simulink model "Longitidunal_Vehicle_Dynamics"  (R2025b)
settings: Solver=ode8  StartTime=0.0  StopTime=200  FixedStep=0.01  RelTol=1e-3
InitFcn:
  | cx=0.32;
  | A=2; %m^2
  | ro=1.22; %kg/m^3
  | r=(15*0.0254)/2+(0.185*0.65); %m
  | rw=0.98*r; %Effectiveradius
  | m=1200; %kg
  | g=9.81; %m/s^2
  | l=2.4; %m
  | a1=1.1; %m
  | a2=1.4; %m
  | h=0.0508; %m
  | mu0=0.015; %Jazar
  | mu1=7e-6; %Jazar
  | mu=0.8; %Jazar
  | teta=0;
  | J_w=1.2; %kg/m^2
  | Iz=3000; %kg/m^2
  | Calfaf=75000; %N/rad
  | Calfar=75000; %N/rad
  | ms=375; %Jazar
  | cs=1200; %Jazar
  | ks=35000; %Jazar
  | mu=75; %Jazar
  | cu=0; %Jazar
  | ku=193000; %
settings Model: Creator=xps  LastModifiedBy=MehrSystem
settings SolverCC: ZeroCrossAlgorithm=Adaptive  AlgebraicLoopSolver=TrustRegion
settings DataIOCC: ReturnWorkspaceOutputs=off
settings OptimizationCC: DefaultParameterBehavior=Inlined  OptimizeBlockIOStorage=off  BufferReuse=off  ReuseModelBlockBuffer=off  GlobalBufferReuse=off  ExpressionFolding=off  EnableMemcpy=off  PassReuseOutputArgsAs=Individual arguments  LocalBlockOutputs=off  ZeroExternalMemoryAtStartup=off  ZeroInternalMemoryAtStartup=off  OptimizeDataStoreBuffers=off  BusAssignmentInplaceUpdate=off  OptimizationLevel=level0  OptimizationCustomize=off  EfficientTunableParamExpr=on
settings DebuggingCC: MaxConsecutiveZCsMsg=none  ParameterTunabilityLossMsg=error  UnconnectedInputMsg=warning  UnconnectedOutputMsg=warning  UnconnectedLineMsg=warning  ArithmeticOperatorsInVariantConditions=warning
settings ModelReferenceCC: EnableRefExpFcnMdlSchedulingChecks=on
settings SFSimCC: SimUseLocalCustomCode=off  MATLABDynamicMemAlloc=off  CustomCodeUndefinedFunction=UseInterfaceOnly
settings RTWCC: SystemTargetFile=ert.tlc  TemplateMakefile=ert_default_tmf  RTWUseLocalCustomCode=off  GPUComputeCapability=3.5  Description=Embedded Coder
settings CodeAppCC: ForceParamTrailComments=on  IgnoreCustomStorageClasses=off  OperatorAnnotations=on  SimulinkDataObjDesc=on  SFDataObjDesc=on  InsertBlockDesc=on
settings ERTTargetCC: ERTCustomFileTemplate=example_file_process.tlc  TargetLangStandard=C99 (ISO)  GenerateSampleERTMain=on  SupportContinuousTime=on

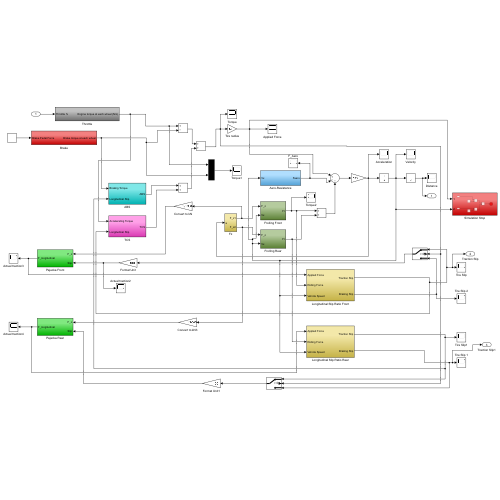
[thumbnail: Simulink's stored preview of the top-level diagram]
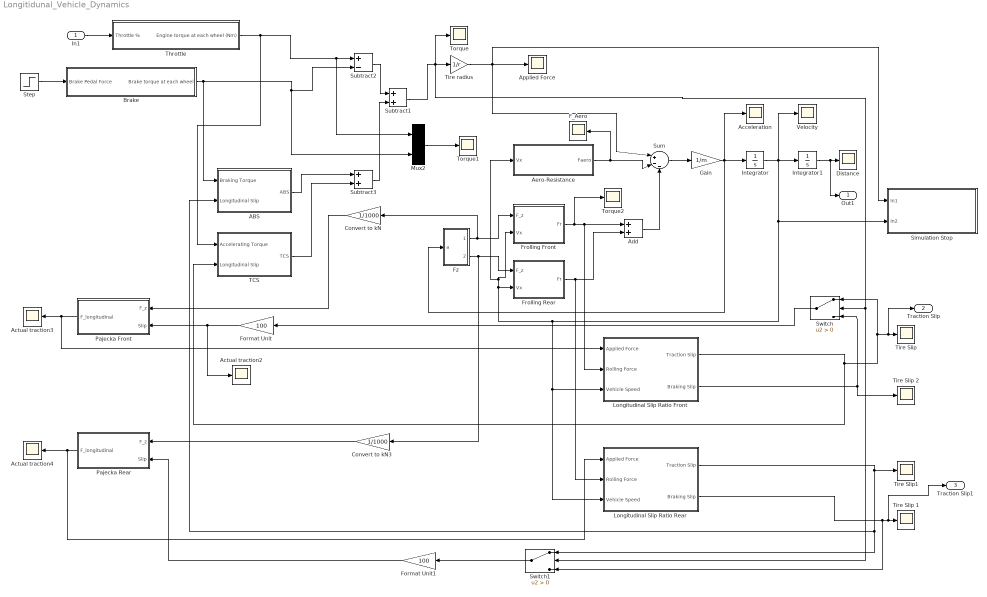
== system Longitidunal_Vehicle_Dynamics ==
  In1 : Inport
  ABS : Subsystem
  Acceleration : Scope
      settings: ActiveDisplayYMinimum=-11.20211075688924  ActiveDisplayYMaximum=1.1595227229876932  DataLoggingVariableName=ScopeData2
  Actual traction2 : Scope
      settings: ActiveDisplayYMinimum=-9.6127540741225162E+14  ActiveDisplayYMaximum=2.5798371932340445E+15  DataLoggingVariableName=ScopeData3
  Actual traction3 : Scope
      settings: ActiveDisplayYMinimum=-2781.3956583754534  ActiveDisplayYMaximum=-2659.1708426364712  DataLoggingVariableName=ScopeData5
  Actual traction4 : Scope
      settings: ActiveDisplayYMinimum=-2116.02176137597  ActiveDisplayYMaximum=-1996.3163945739989  DataLoggingVariableName=ScopeData2
  Add : Sum
  Aero-Resistance : Subsystem
  Applied Force : Scope
      settings: ActiveDisplayYMinimum=-7916.33146  ActiveDisplayYMaximum=1737.7313  DataLoggingVariableName=ScopeData6
  Brake : Subsystem
  Convert to kN : Gain  Gain=1/1000
  Convert to kN3 : Gain  Gain=1/1000
  Distance : Scope
      settings: ActiveDisplayYMinimum=-2186.3043007629622  ActiveDisplayYMaximum=242.92270008477351
  F_Aero : Scope
      settings: ActiveDisplayYMinimum=-66.76965  ActiveDisplayYMaximum=600.92681
  Format Unit : Gain  Gain=100
  Format Unit1 : Gain  Gain=100
  Frolling Front : Subsystem
  Frolling Rear : Subsystem
  Fz : Subsystem
  Gain : Gain  Gain=1/m
  Integrator : Integrator
  Integrator1 : Integrator
  Longitudinal Slip Ratio Front : Subsystem
  Longitudinal Slip Ratio Rear : Subsystem
  Mux2 : Mux  Inputs=2
  Pajecka Front : Subsystem
  Pajecka Rear : Subsystem
  Simulation Stop : Subsystem
  Step : Step  Time=120  After=30  SampleTime=0
  Subtract1 : Sum
  Subtract2 : Sum  Inputs=+-
  Subtract3 : Sum
  Sum : Sum  Inputs=|+--
  Switch : Switch  Criteria=u2 > Threshold  SaturateOnIntegerOverflow=off  InputSameDT=off
  Switch1 : Switch  Criteria=u2 > Threshold  SaturateOnIntegerOverflow=off  InputSameDT=off
  TCS : Subsystem
  Throttle : Subsystem
  Tire Slip : Scope
      settings: ActiveDisplayYMinimum=0.99985  ActiveDisplayYMaximum=1.00139  DataLoggingVariableName=ScopeData2
  Tire Slip 1 : Scope
      settings: ActiveDisplayYMinimum=-592.75065171892868  ActiveDisplayYMaximum=58.517501440809937  DataLoggingVariableName=ScopeData6
  Tire Slip 2 : Scope
      settings: ActiveDisplayYMinimum=-1469.7388232940821  ActiveDisplayYMaximum=-771.732664711504  DataLoggingVariableName=ScopeData3
  Tire Slip1 : Scope
      settings: ActiveDisplayYMinimum=0.98434  ActiveDisplayYMaximum=1.14093  DataLoggingVariableName=ScopeData7
  Tire radius : Gain  Gain=1/r
  Torque : Scope
      settings: ActiveDisplayYMinimum=-220  ActiveDisplayYMaximum=-20  DataLoggingVariableName=ScopeData5
  Torque1 : Scope
      settings: ActiveDisplayYMinimum=-75  ActiveDisplayYMaximum=675
  Torque2 : Scope
      settings: ActiveDisplayYMinimum=33.8504  ActiveDisplayYMaximum=141.74668  DataLoggingVariableName=ScopeData2
  Velocity : Scope
      settings: ActiveDisplayYMinimum=-4.60487  ActiveDisplayYMaximum=41.44379
  Out1 : Outport
  Traction Slip : Outport  Port=2
  Traction Slip1 : Outport  Port=3
  wires:
  Gain/1 -> Fz/1(a), Acceleration/1, Integrator/1
  Integrator/1 -> Simulation Stop/2(In2), Longitudinal Slip Ratio Rear/3(Vehicle Speed), Longitudinal Slip Ratio Front/3(Vehicle Speed), Aero-Resistance/1(Vx), Frolling Front/2(Vx), Frolling Rear/2(Vx), Velocity/1, Integrator1/1
  Sum/1 -> Gain/1
  Aero-Resistance/1(Faero) -> F_Aero/1, Sum/2
  Fz/1(F_z1) -> Convert to kN/1, Frolling Front/1(F_z)
  Fz/2(F_z2) -> Convert to kN3/1, Frolling Rear/1(F_z)
  Frolling Front/1(Fr) -> Torque2/1, Longitudinal Slip Ratio Front/2(Rolling Force), Add/1
  Add/1 -> Sum/3
  Subtract1/1 -> Torque/1, Switch/2, Switch1/2, Tire radius/1
  Throttle/1(Engine torque at each wheel (Nm)) -> TCS/1(Accelerating Torque), Subtract2/1, Mux2/1
  Brake/1(Brake torque at each wheel) -> Subtract2/2, Mux2/2, ABS/1(Braking Torque)
  Integrator1/1 -> Out1/1, Distance/1
  Convert to kN/1 -> Pajecka Front/1(F_z)
  Format Unit/1 -> Pajecka Front/2(Slip), Actual traction2/1
  Longitudinal Slip Ratio Front/1(Traction Slip) -> TCS/2(Longitudinal Slip), Switch/1, Traction Slip/1, Tire Slip/1
  Longitudinal Slip Ratio Front/2(Braking Slip) -> Switch/3, Tire Slip 2/1
  Longitudinal Slip Ratio Rear/2(Braking Slip) -> Switch1/3, Traction Slip1/1, Tire Slip 1/1
  Convert to kN3/1 -> Pajecka Rear/1(F_z)
  Longitudinal Slip Ratio Rear/1(Traction Slip) -> ABS/2(Longitudinal Slip), Switch1/1, Tire Slip1/1
  Pajecka Rear/1(F_longitudinal) -> Longitudinal Slip Ratio Rear/1(Applied Force), Actual traction4/1
  Switch/1 -> Format Unit/1
  Switch1/1 -> Format Unit1/1
  Mux2/1 -> Torque1/1
  In1/1 -> Throttle/1(Throttle %)
  Format Unit1/1 -> Pajecka Rear/2(Slip)
  Tire radius/1 -> Simulation Stop/1(In1), Sum/1, Applied Force/1
  Step/1 -> Brake/1(Brake Pedal Force)
  Pajecka Front/1(F_longitudinal) -> Actual traction3/1, Longitudinal Slip Ratio Front/1(Applied Force)
  Subtract2/1 -> Subtract1/1
  Frolling Rear/1(Fr) -> Longitudinal Slip Ratio Rear/2(Rolling Force), Add/2
  TCS/1(TCS) -> Subtract3/2
  ABS/1(ABS) -> Subtract3/1
  Subtract3/1 -> Subtract1/2

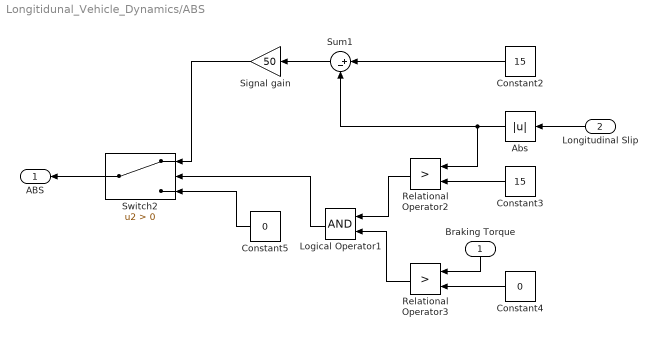
== system Longitidunal_Vehicle_Dynamics/ABS ==
  Braking Torque : Inport
  Longitudinal Slip : Inport  Port=2
  Abs : Abs  SaturateOnIntegerOverflow=off
  Constant2 : Constant  Value=15
  Constant3 : Constant  Value=15
  Constant4 : Constant  Value=0
  Constant5 : Constant  Value=0
  Logical Operator1 : Logic  AllPortsSameDT=off  OutDataTypeStr=boolean
  Relational Operator2 : RelationalOperator  Operator=>  OutDataTypeStr=boolean  RndMeth=Simplest  InputSameDT=off
  Relational Operator3 : RelationalOperator  Operator=>  OutDataTypeStr=boolean  RndMeth=Simplest  InputSameDT=off
  Signal gain : Gain  Gain=50
  Sum1 : Sum  Inputs=|+-
  Switch2 : Switch  Criteria=u2 > Threshold  SaturateOnIntegerOverflow=off  InputSameDT=off
  ABS : Outport  VectorParamsAs1DForOutWhenUnconnected=off
  wires:
  Sum1/1 -> Signal gain/1
  Constant4/1 -> Relational Operator3/2
  Longitudinal Slip/1 -> Abs/1
  Braking Torque/1 -> Relational Operator3/1
  Switch2/1 -> ABS/1
  Relational Operator2/1 -> Logical Operator1/1
  Constant3/1 -> Relational Operator2/2
  Logical Operator1/1 -> Switch2/2
  Constant2/1 -> Sum1/1
  Relational Operator3/1 -> Logical Operator1/2
  Constant5/1 -> Switch2/3
  Abs/1 -> Relational Operator2/1, Sum1/2
  Signal gain/1 -> Switch2/1

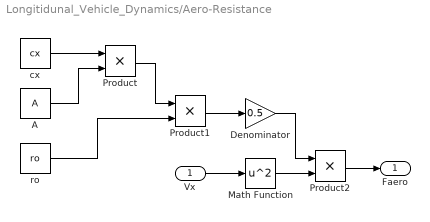
== system Longitidunal_Vehicle_Dynamics/Aero-Resistance ==
  Vx : Inport
  A : Constant  Value=A
  Denominator : Gain  Gain=0.5
  Math Function : Math  Operator=square  SignedPower=on
  Product : Product
  Product1 : Product
  Product2 : Product
  cx : Constant  Value=cx
  ro : Constant  Value=ro
  Faero : Outport  VectorParamsAs1DForOutWhenUnconnected=off
  wires:
  A/1 -> Product/2
  Product1/1 -> Denominator/1
  Denominator/1 -> Product2/1
  Vx/1 -> Math Function/1
  Product2/1 -> Faero/1
  ro/1 -> Product1/2
  cx/1 -> Product/1
  Math Function/1 -> Product2/2
  Product/1 -> Product1/1

== system Longitidunal_Vehicle_Dynamics/Brake ==
  Brake Pedal Force : Inport
  Gain : Gain  Gain=400
  Gain1 : Gain
  r_static : Gain  Gain=0.3
  Brake torque at each wheel : Outport  VectorParamsAs1DForOutWhenUnconnected=off
  wires:
  Gain1/1 -> r_static/1
  Gain/1 -> Gain1/1
  Brake Pedal Force/1 -> Gain/1
  r_static/1 -> Brake torque at each wheel/1

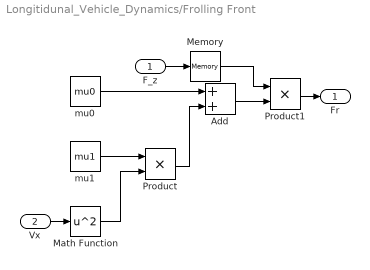
== system Longitidunal_Vehicle_Dynamics/Frolling Front ==
  F_z : Inport
  Vx : Inport  Port=2
  Add : Sum
  Math Function : Math  Operator=square  SignedPower=on
  Memory : Memory
  Product : Product
  Product1 : Product
  mu0 : Constant  Value=mu0
  mu1 : Constant  Value=mu1
  Fr : Outport  VectorParamsAs1DForOutWhenUnconnected=off
  wires:
  Add/1 -> Product1/2
  Math Function/1 -> Product/2
  Product/1 -> Add/2
  mu0/1 -> Add/1
  mu1/1 -> Product/1
  Vx/1 -> Math Function/1
  Product1/1 -> Fr/1
  F_z/1 -> Memory/1
  Memory/1 -> Product1/1

== system Longitidunal_Vehicle_Dynamics/Frolling Rear ==
  F_z : Inport
  Vx : Inport  Port=2
  Add : Sum
  Math Function : Math  Operator=square  SignedPower=on
  Memory : Memory
  Product : Product
  Product1 : Product
  mu0 : Constant  Value=mu0
  mu1 : Constant  Value=mu1
  Fr : Outport  VectorParamsAs1DForOutWhenUnconnected=off
  wires:
  F_z/1 -> Memory/1
  Product1/1 -> Fr/1
  Vx/1 -> Math Function/1
  mu1/1 -> Product/1
  mu0/1 -> Add/1
  Product/1 -> Add/2
  Math Function/1 -> Product/2
  Add/1 -> Product1/2
  Memory/1 -> Product1/1

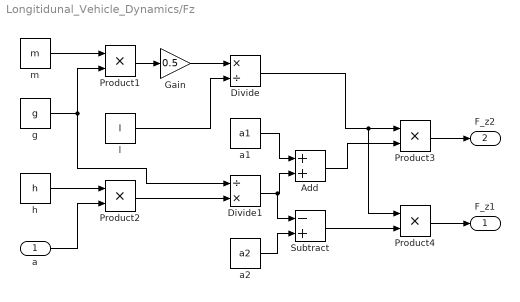
== system Longitidunal_Vehicle_Dynamics/Fz ==
  a : Inport
  Add : Sum
  Divide : Product  Inputs=*/
  Divide1 : Product  Inputs=/*
  Gain : Gain  Gain=0.5
  Product{1..4} (4 alike) : Product
  Subtract : Sum  Inputs=-+
  a1 : Constant  Value=a1
  a2 : Constant  Value=a2
  g : Constant  Value=g
  h : Constant  Value=h
  l : Constant  Value=l
  m : Constant  Value=m
  F_z1 : Outport  VectorParamsAs1DForOutWhenUnconnected=off
  F_z2 : Outport  Port=2  VectorParamsAs1DForOutWhenUnconnected=off
  wires:
  m/1 -> Product1/1
  g/1 -> Divide1/1, Product1/2
  Product1/1 -> Gain/1
  Gain/1 -> Divide/1
  l/1 -> Divide/2
  h/1 -> Product2/1
  Product2/1 -> Divide1/2
  a1/1 -> Add/1
  Divide1/1 -> Subtract/1, Add/2
  Divide/1 -> Product4/1, Product3/1
  Add/1 -> Product3/2
  a2/1 -> Subtract/2
  Subtract/1 -> Product4/2
  Product4/1 -> F_z1/1
  Product3/1 -> F_z2/1
  a/1 -> Product2/2

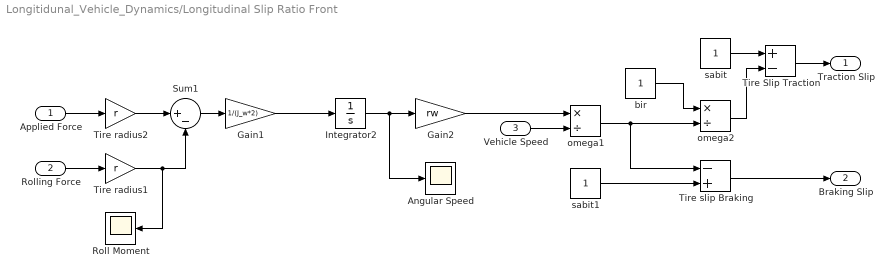
== system Longitidunal_Vehicle_Dynamics/Longitudinal Slip Ratio Front ==
  Applied Force : Inport
  Rolling Force : Inport  Port=2
  Vehicle Speed : Inport  Port=3
  Angular Speed : Scope
      settings: ActiveDisplayYMinimum=-754.25402  ActiveDisplayYMaximum=6788.28715
  Gain1 : Gain  Gain=1/(J_w*2)
  Gain2 : Gain  Gain=rw
  Integrator2 : Integrator  InitialCondition=0.0001
  Roll Moment : Scope
      settings: ActiveDisplayYMinimum=12.74052  ActiveDisplayYMaximum=24.56596  DataLoggingVariableName=ScopeData6
  Sum1 : Sum  Inputs=|+-
  Tire Slip Traction : Sum  Inputs=+-
  Tire radius1 : Gain  Gain=r
  Tire radius2 : Gain  Gain=r
  Tire slip Braking : Sum  Inputs=-+
  bir : Constant
  omega1 : Product  Inputs=*/
  omega2 : Product  Inputs=*/
  sabit : Constant
  sabit1 : Constant
  Traction Slip : Outport  VectorParamsAs1DForOutWhenUnconnected=off
  Braking Slip : Outport  Port=2  VectorParamsAs1DForOutWhenUnconnected=off
  wires:
  Rolling Force/1 -> Tire radius1/1
  Vehicle Speed/1 -> omega1/2
  Tire slip Braking/1 -> Braking Slip/1
  Integrator2/1 -> Gain2/1, Angular Speed/1
  sabit/1 -> Tire Slip Traction/1
  bir/1 -> omega2/1
  omega2/1 -> Tire Slip Traction/2
  Tire Slip Traction/1 -> Traction Slip/1
  Gain1/1 -> Integrator2/1
  Gain2/1 -> omega1/1
  omega1/1 -> Tire slip Braking/1, omega2/2
  Tire radius1/1 -> Sum1/2, Roll Moment/1
  sabit1/1 -> Tire slip Braking/2
  Applied Force/1 -> Tire radius2/1
  Sum1/1 -> Gain1/1
  Tire radius2/1 -> Sum1/1

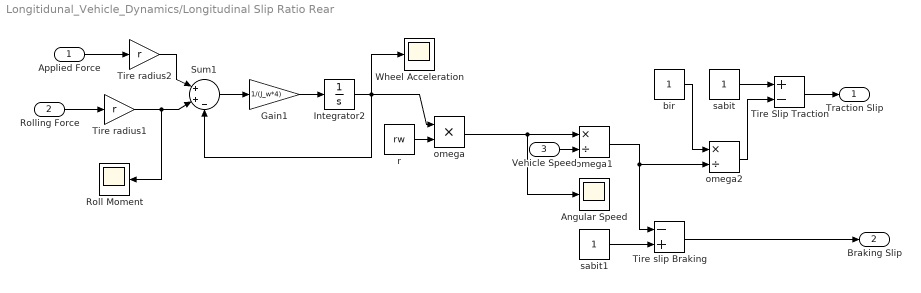
== system Longitidunal_Vehicle_Dynamics/Longitudinal Slip Ratio Rear ==
  Applied Force : Inport
  Rolling Force : Inport  Port=2
  Vehicle Speed : Inport  Port=3
  Angular Speed : Scope
      settings: ActiveDisplayYMinimum=-1  ActiveDisplayYMaximum=1
  Gain1 : Gain  Gain=1/(J_w*4)
  Integrator2 : Integrator  InitialCondition=0.0001
  Roll Moment : Scope
      settings: ActiveDisplayYMinimum=9.72165  ActiveDisplayYMaximum=18.82881  DataLoggingVariableName=ScopeData6
  Sum1 : Sum  Inputs=|++-
  Tire Slip Traction : Sum  Inputs=+-
  Tire radius1 : Gain  Gain=r
  Tire radius2 : Gain  Gain=r
  Tire slip Braking : Sum  Inputs=-+
  Wheel Acceleration : Scope
      settings: ActiveDisplayYMinimum=-31.80693  ActiveDisplayYMaximum=286.2624  DataLoggingVariableName=ScopeData4
  bir : Constant
  omega : Product  Inputs=**
  omega1 : Product  Inputs=*/
  omega2 : Product  Inputs=*/
  r : Constant  Value=rw
  sabit : Constant
  sabit1 : Constant
  Traction Slip : Outport  VectorParamsAs1DForOutWhenUnconnected=off
  Braking Slip : Outport  Port=2  VectorParamsAs1DForOutWhenUnconnected=off
  wires:
  sabit1/1 -> Tire slip Braking/2
  Tire radius1/1 -> Roll Moment/1, Sum1/2
  omega1/1 -> omega2/2, Tire slip Braking/1
  omega/1 -> omega1/1, Angular Speed/1
  r/1 -> omega/2
  Gain1/1 -> Integrator2/1
  Tire Slip Traction/1 -> Traction Slip/1
  omega2/1 -> Tire Slip Traction/2
  bir/1 -> omega2/1
  Sum1/1 -> Gain1/1
  sabit/1 -> Tire Slip Traction/1
  Integrator2/1 -> Sum1/3, Wheel Acceleration/1, omega/1
  Tire slip Braking/1 -> Braking Slip/1
  Vehicle Speed/1 -> omega1/2
  Applied Force/1 -> Tire radius2/1
  Rolling Force/1 -> Tire radius1/1
  Tire radius2/1 -> Sum1/1

== system Longitidunal_Vehicle_Dynamics/Pajecka Front ==
  F_z : Inport
  Slip : Inport  Port=2
  Longitudinal : Subsystem
  Subsystem : Subsystem
  F_longitudinal : Outport  VectorParamsAs1DForOutWhenUnconnected=off
  wires:
  Longitudinal/1(F) -> F_longitudinal/1
  F_z/1 -> Subsystem/1(F_z)
  Slip/1 -> Subsystem/2(slip)
  Subsystem/4(E) -> Longitudinal/3(E)
  Subsystem/5(Bx1) -> Longitudinal/4(Bx1)
  Subsystem/1(C) -> Longitudinal/1(C)
  Subsystem/2(D) -> Longitudinal/2(D)
  Subsystem/3(V) -> Longitudinal/5(V)

== system Longitidunal_Vehicle_Dynamics/Pajecka Rear ==
  F_z : Inport
  Slip : Inport  Port=2
  Longitudinal : Subsystem
  Subsystem : Subsystem
  F_longitudinal : Outport  VectorParamsAs1DForOutWhenUnconnected=off
  wires:
  Longitudinal/1(F) -> F_longitudinal/1
  F_z/1 -> Subsystem/1(F_z)
  Slip/1 -> Subsystem/2(slip)
  Subsystem/4(E) -> Longitudinal/3(E)
  Subsystem/5(Bx1) -> Longitudinal/4(Bx1)
  Subsystem/1(C) -> Longitudinal/1(C)
  Subsystem/2(D) -> Longitudinal/2(D)
  Subsystem/3(V) -> Longitudinal/5(V)

== system Longitidunal_Vehicle_Dynamics/Simulation Stop ==
  In1 : Inport
  In2 : Inport  Port=2
  Constant : Constant  Value=0.1
  Constant1 : Constant  Value=0
  Logical Operator : Logic  AllPortsSameDT=off  OutDataTypeStr=boolean
  Relational Operator : RelationalOperator  Operator=<=  OutDataTypeStr=boolean  RndMeth=Simplest  InputSameDT=off
  Relational Operator1 : RelationalOperator  Operator=<  OutDataTypeStr=boolean  RndMeth=Simplest  InputSameDT=off
  Stop Simulation : Stop
  wires:
  Relational Operator1/1 -> Logical Operator/1
  Relational Operator/1 -> Logical Operator/2
  Constant/1 -> Relational Operator/2
  Constant1/1 -> Relational Operator1/2
  Logical Operator/1 -> Stop Simulation/1
  In2/1 -> Relational Operator/1
  In1/1 -> Relational Operator1/1

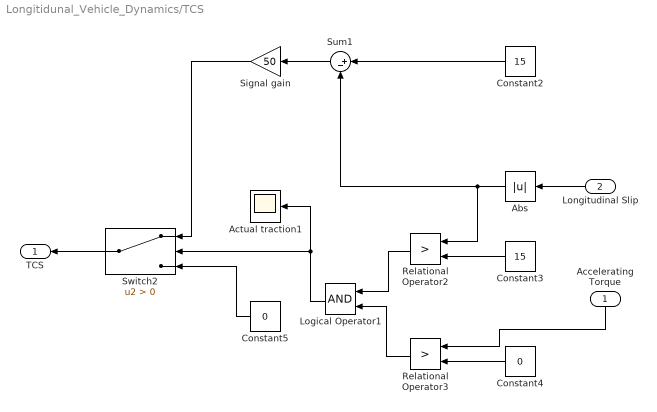
== system Longitidunal_Vehicle_Dynamics/TCS ==
  Accelerating Torque : Inport
  Longitudinal Slip : Inport  Port=2
  Abs : Abs  SaturateOnIntegerOverflow=off
  Actual traction1 : Scope
      settings: ActiveDisplayYMinimum=-1  ActiveDisplayYMaximum=1
  Constant2 : Constant  Value=15
  Constant3 : Constant  Value=15
  Constant4 : Constant  Value=0
  Constant5 : Constant  Value=0
  Logical Operator1 : Logic  AllPortsSameDT=off  OutDataTypeStr=boolean
  Relational Operator2 : RelationalOperator  Operator=>  OutDataTypeStr=boolean  RndMeth=Simplest  InputSameDT=off
  Relational Operator3 : RelationalOperator  Operator=>  OutDataTypeStr=boolean  RndMeth=Simplest  InputSameDT=off
  Signal gain : Gain  Gain=50
  Sum1 : Sum  Inputs=|+-
  Switch2 : Switch  Criteria=u2 > Threshold  SaturateOnIntegerOverflow=off  InputSameDT=off
  TCS : Outport  VectorParamsAs1DForOutWhenUnconnected=off
  wires:
  Signal gain/1 -> Switch2/1
  Abs/1 -> Sum1/2, Relational Operator2/1
  Constant5/1 -> Switch2/3
  Relational Operator3/1 -> Logical Operator1/2
  Constant2/1 -> Sum1/1
  Logical Operator1/1 -> Actual traction1/1, Switch2/2
  Constant3/1 -> Relational Operator2/2
  Relational Operator2/1 -> Logical Operator1/1
  Switch2/1 -> TCS/1
  Accelerating Torque/1 -> Relational Operator3/1
  Longitudinal Slip/1 -> Abs/1
  Constant4/1 -> Relational Operator3/2
  Sum1/1 -> Signal gain/1

== system Longitidunal_Vehicle_Dynamics/Throttle ==
  Throttle % : Inport
  Gain : Gain  Gain=2.4
  Gain1 : Gain
  Engine torque at each wheel (Nm) : Outport  VectorParamsAs1DForOutWhenUnconnected=off
  wires:
  Gain/1 -> Gain1/1
  Throttle %/1 -> Gain/1
  Gain1/1 -> Engine torque at each wheel (Nm)/1

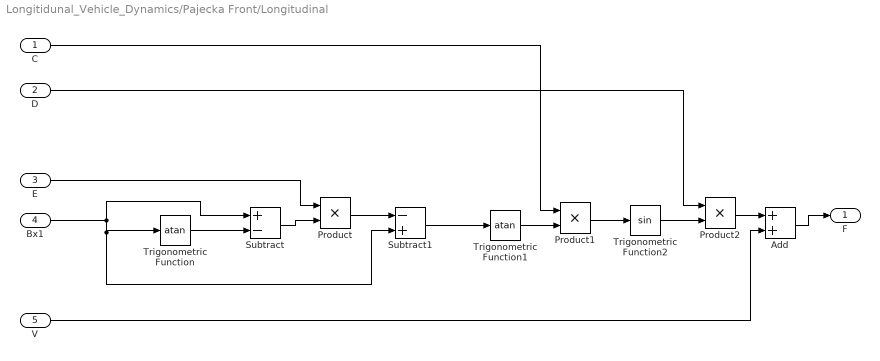
== system Longitidunal_Vehicle_Dynamics/Pajecka Front/Longitudinal ==
  C : Inport
  D : Inport  Port=2
  E : Inport  Port=3
  Bx1 : Inport  Port=4
  V : Inport  Port=5
  Add : Sum
  Product : Product
  Product1 : Product
  Product2 : Product
  Subtract : Sum  Inputs=+-
  Subtract1 : Sum  Inputs=-+
  Trigonometric Function : Trigonometry  Operator=atan
  Trigonometric Function1 : Trigonometry  Operator=atan
  Trigonometric Function2 : Trigonometry
  F : Outport  VectorParamsAs1DForOutWhenUnconnected=off
  wires:
  Subtract/1 -> Product/2
  Trigonometric Function/1 -> Subtract/2
  Product/1 -> Subtract1/1
  Trigonometric Function1/1 -> Product1/2
  D/1 -> Product2/1
  Product1/1 -> Trigonometric Function2/1
  Trigonometric Function2/1 -> Product2/2
  Bx1/1 -> Trigonometric Function/1, Subtract1/2, Subtract/1
  Subtract1/1 -> Trigonometric Function1/1
  E/1 -> Product/1
  C/1 -> Product1/1
  Product2/1 -> Add/1
  V/1 -> Add/2
  Add/1 -> F/1

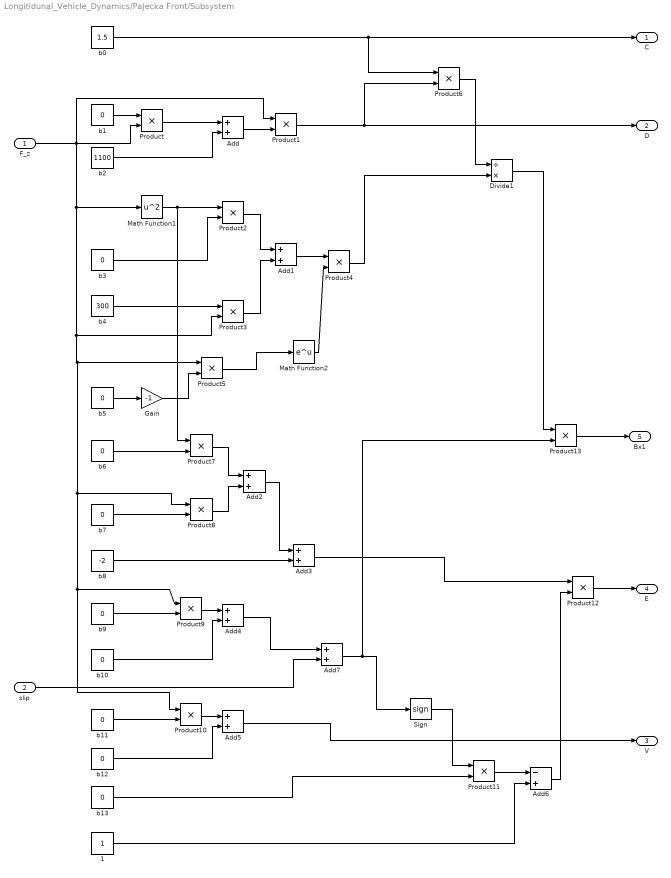
== system Longitidunal_Vehicle_Dynamics/Pajecka Front/Subsystem ==
  F_z : Inport
  slip : Inport  Port=2
  1 : Constant
  Add{,1..5,7} (7 alike) : Sum
  Add6 : Sum  Inputs=-+
  Divide1 : Product  Inputs=/*
  Gain : Gain  Gain=-1
  Math Function1 : Math  Operator=square  SignedPower=on
  Math Function2 : Math  SignedPower=on
  Product{,1..13} (14 alike) : Product
  Sign : Signum
  b0 : Constant  Value=1.5
  b{1,3,5..7,9..13} (10 alike) : Constant  Value=0
  b2 : Constant  Value=1100
  b4 : Constant  Value=300
  b8 : Constant  Value=-2
  C : Outport  VectorParamsAs1DForOutWhenUnconnected=off
  D : Outport  Port=2  VectorParamsAs1DForOutWhenUnconnected=off
  V : Outport  Port=3  VectorParamsAs1DForOutWhenUnconnected=off
  E : Outport  Port=4  VectorParamsAs1DForOutWhenUnconnected=off
  Bx1 : Outport  Port=5  VectorParamsAs1DForOutWhenUnconnected=off
  wires:
  Add3/1 -> Product12/1
  Add1/1 -> Product4/1
  1/1 -> Add6/2
  b13/1 -> Product11/2
  slip/1 -> Add7/2
  Product12/1 -> E/1
  Product2/1 -> Add1/1
  Sign/1 -> Product11/1
  Add7/1 -> Product13/2, Sign/1
  Math Function2/1 -> Product4/2
  b6/1 -> Product7/2
  Product13/1 -> Bx1/1
  Product11/1 -> Add6/1
  b12/1 -> Add5/2
  b10/1 -> Add4/2
  b8/1 -> Add3/2
  b7/1 -> Product8/2
  Add6/1 -> Product12/2
  Product9/1 -> Add4/1
  Product4/1 -> Divide1/2
  Math Function1/1 -> Product7/1, Product2/1
  b0/1 -> C/1, Product6/1
  b2/1 -> Add/2
  Add5/1 -> V/1
  b9/1 -> Product9/2
  b1/1 -> Product/1
  F_z/1 -> Product3/2, Product10/1, Product9/1, Product8/1, Product5/1, Math Function1/1, Product1/1, Product/2
  Product/1 -> Add/1
  Gain/1 -> Product5/2
  Divide1/1 -> Product13/1
  b4/1 -> Product3/1
  Add/1 -> Product1/2
  Add4/1 -> Add7/1
  Product10/1 -> Add5/1
  Product5/1 -> Math Function2/1
  Add2/1 -> Add3/1
  Product6/1 -> Divide1/1
  b5/1 -> Gain/1
  Product8/1 -> Add2/2
  Product7/1 -> Add2/1
  Product3/1 -> Add1/2
  b3/1 -> Product2/2
  b11/1 -> Product10/2
  Product1/1 -> D/1, Product6/2

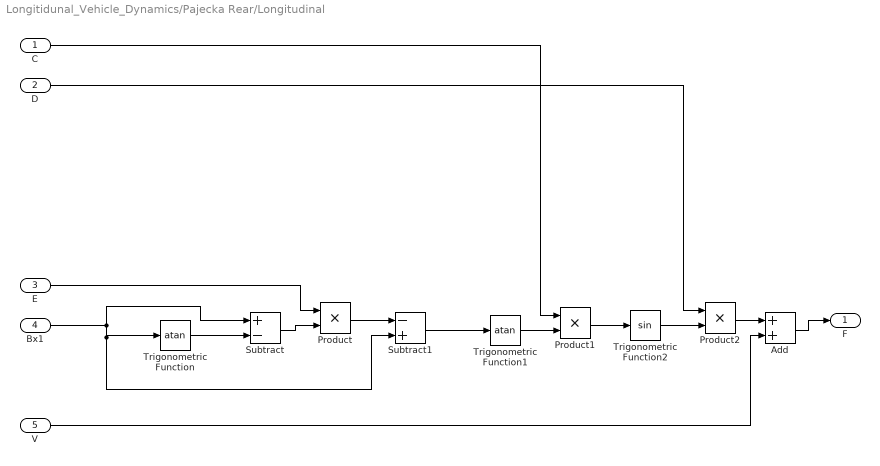
== system Longitidunal_Vehicle_Dynamics/Pajecka Rear/Longitudinal ==
  C : Inport
  D : Inport  Port=2
  E : Inport  Port=3
  Bx1 : Inport  Port=4
  V : Inport  Port=5
  Add : Sum
  Product : Product
  Product1 : Product
  Product2 : Product
  Subtract : Sum  Inputs=+-
  Subtract1 : Sum  Inputs=-+
  Trigonometric Function : Trigonometry  Operator=atan
  Trigonometric Function1 : Trigonometry  Operator=atan
  Trigonometric Function2 : Trigonometry
  F : Outport  VectorParamsAs1DForOutWhenUnconnected=off
  wires:
  Subtract/1 -> Product/2
  Trigonometric Function/1 -> Subtract/2
  Product/1 -> Subtract1/1
  Trigonometric Function1/1 -> Product1/2
  D/1 -> Product2/1
  Product1/1 -> Trigonometric Function2/1
  Trigonometric Function2/1 -> Product2/2
  Bx1/1 -> Trigonometric Function/1, Subtract1/2, Subtract/1
  Subtract1/1 -> Trigonometric Function1/1
  E/1 -> Product/1
  C/1 -> Product1/1
  Product2/1 -> Add/1
  V/1 -> Add/2
  Add/1 -> F/1

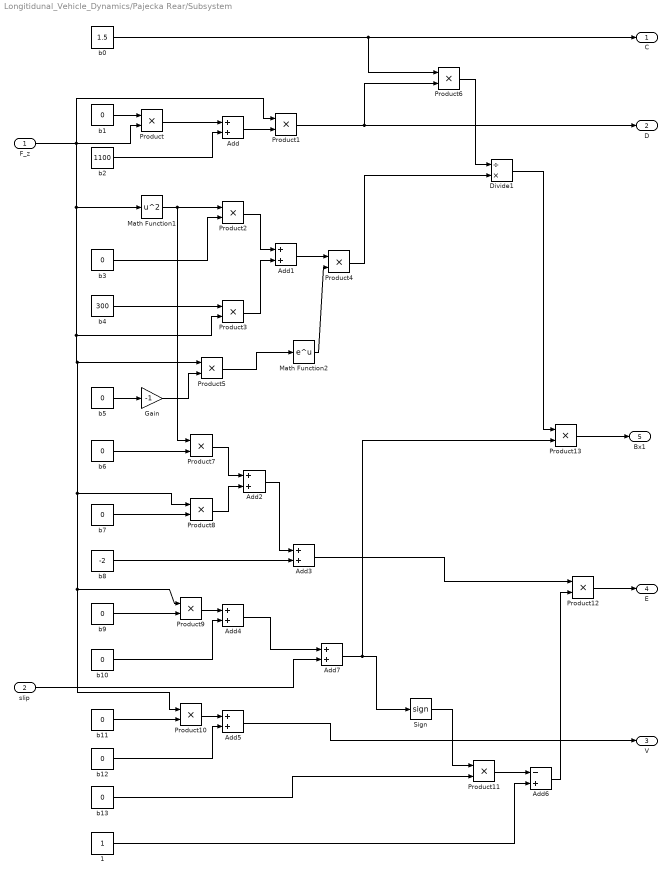
== system Longitidunal_Vehicle_Dynamics/Pajecka Rear/Subsystem ==
  F_z : Inport
  slip : Inport  Port=2
  1 : Constant
  Add{,1..5,7} (7 alike) : Sum
  Add6 : Sum  Inputs=-+
  Divide1 : Product  Inputs=/*
  Gain : Gain  Gain=-1
  Math Function1 : Math  Operator=square  SignedPower=on
  Math Function2 : Math  SignedPower=on
  Product{,1..13} (14 alike) : Product
  Sign : Signum
  b0 : Constant  Value=1.5
  b{1,3,5..7,9..13} (10 alike) : Constant  Value=0
  b2 : Constant  Value=1100
  b4 : Constant  Value=300
  b8 : Constant  Value=-2
  C : Outport  VectorParamsAs1DForOutWhenUnconnected=off
  D : Outport  Port=2  VectorParamsAs1DForOutWhenUnconnected=off
  V : Outport  Port=3  VectorParamsAs1DForOutWhenUnconnected=off
  E : Outport  Port=4  VectorParamsAs1DForOutWhenUnconnected=off
  Bx1 : Outport  Port=5  VectorParamsAs1DForOutWhenUnconnected=off
  wires:
  Add3/1 -> Product12/1
  Add1/1 -> Product4/1
  1/1 -> Add6/2
  b13/1 -> Product11/2
  slip/1 -> Add7/2
  Product12/1 -> E/1
  Product2/1 -> Add1/1
  Sign/1 -> Product11/1
  Add7/1 -> Product13/2, Sign/1
  Math Function2/1 -> Product4/2
  b6/1 -> Product7/2
  Product13/1 -> Bx1/1
  Product11/1 -> Add6/1
  b12/1 -> Add5/2
  b10/1 -> Add4/2
  b8/1 -> Add3/2
  b7/1 -> Product8/2
  Add6/1 -> Product12/2
  Product9/1 -> Add4/1
  Product4/1 -> Divide1/2
  Math Function1/1 -> Product7/1, Product2/1
  b0/1 -> C/1, Product6/1
  b2/1 -> Add/2
  Add5/1 -> V/1
  b9/1 -> Product9/2
  b1/1 -> Product/1
  F_z/1 -> Product3/2, Product10/1, Product9/1, Product8/1, Product5/1, Math Function1/1, Product1/1, Product/2
  Product/1 -> Add/1
  Gain/1 -> Product5/2
  Divide1/1 -> Product13/1
  b4/1 -> Product3/1
  Add/1 -> Product1/2
  Add4/1 -> Add7/1
  Product10/1 -> Add5/1
  Product5/1 -> Math Function2/1
  Add2/1 -> Add3/1
  Product6/1 -> Divide1/1
  b5/1 -> Gain/1
  Product8/1 -> Add2/2
  Product7/1 -> Add2/1
  Product3/1 -> Add1/2
  b3/1 -> Product2/2
  b11/1 -> Product10/2
  Product1/1 -> D/1, Product6/2
